simulink model "Modulpruefstand_sim"  (R2024a)
settings: Solver=ode4  StartTime=0.0  StopTime=2  FixedStep=T_A  RelTol=1e-3  EnableMultiTasking=on
values from neighbouring files (symbols this model uses):
  b_Reib = 0    [Modulpruefstand.m]
  g = 9.81    [Modulpruefstand.m]
  I_qstart = 0    [Modulpruefstand.m]
  J = 1.385e-5    (= 1.385e-05)    [Modulpruefstand.m]
  J_Last = m_Last*l_Last^2/(N^2)    (= 0)    [Modulpruefstand.m]
  Ki_I = V_IR/T_In    (= 48205)    [Modulpruefstand.m]
  Ki_omega = V_omegaR/T_omegan    (= 257.626488095)    [Modulpruefstand.m]
  Ki_phi = V_phiR/T_phin    (= 195312.5)    [Modulpruefstand.m]
  Kp_I = V_IR    (= 32.515)    [Modulpruefstand.m]
  Kp_omega = V_omegaR    (= 0.206101190476)    [Modulpruefstand.m]
  Kp_phi = V_phiR    (= 625)    [Modulpruefstand.m]
  l_Last = 0.3    [Modulpruefstand.m]
  L_q = 6.503e-3    (= 0.006503)    [Modulpruefstand.m]
  m_Last = 0    [Modulpruefstand.m]
  Messrauschen = true    [Modulpruefstand.m]
  N = 100    [Modulpruefstand.m]
  n_abs = 2^(17)    (= 131072)    [Modulpruefstand.m]
  n_ink = 11520    [Modulpruefstand.m]
  omega_mstart = 0    [Modulpruefstand.m]
  p = 4    [Modulpruefstand.m]
  phi_mstart = 0    [Modulpruefstand.m]
  psi_PM = 0.028    [Modulpruefstand.m]
  R = 9.641    [Modulpruefstand.m]
  r_abs = 3.77e-5    (= 3.77e-05)    [Modulpruefstand.m]
  r_ink = 1e-5    (= 1e-05)    [Modulpruefstand.m]
  r_strom = 1e-9    (= 1e-09)    [Modulpruefstand.m]
  Signaltyp = 2    [Modulpruefstand.m]
  T_A = 1e-5    (= 1e-05)    [Modulpruefstand.m]
  T_LV = 1e-4    (= 0.0001)    [Modulpruefstand.m]
  T_omegaTP = 10*T_A    (= 0.0001)    [Modulpruefstand.m]
  U_max = 100    [Modulpruefstand.m]
undefined symbols (not defined in the file or in its folder): Kd_strom
libraries: simulink x5, slpidlib x3
settings Model: Creator=ga25cah  LastModifiedBy=75737
settings SolverCC: AlgebraicLoopSolver=TrustRegion
settings DataIOCC: SaveOutput=off  SignalLogging=off  DSMLogging=off  ReturnWorkspaceOutputs=off  TimeSaveName=t_sim
settings DebuggingCC: UnconnectedInputMsg=warning  UnconnectedOutputMsg=warning  UnconnectedLineMsg=warning  ArithmeticOperatorsInVariantConditions=warning
settings ModelReferenceCC: EnableRefExpFcnMdlSchedulingChecks=on
settings SFSimCC: SimUseLocalCustomCode=off  CustomCodeUndefinedFunction=UseInterfaceOnly
settings RTWCC: RTWUseLocalCustomCode=off  GPUComputeCapability=3.5
settings CodeAppCC: StateflowObjectComments=on

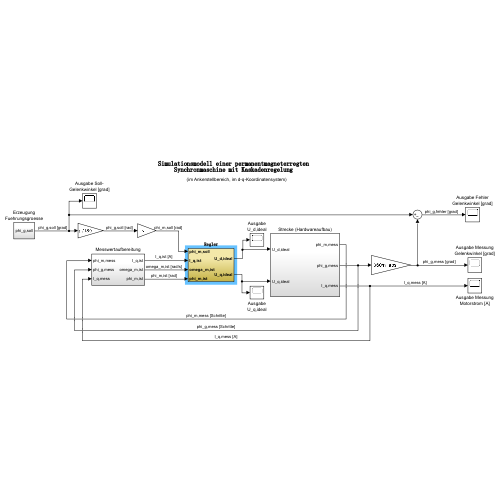
[thumbnail: Simulink's stored preview of the top-level diagram]
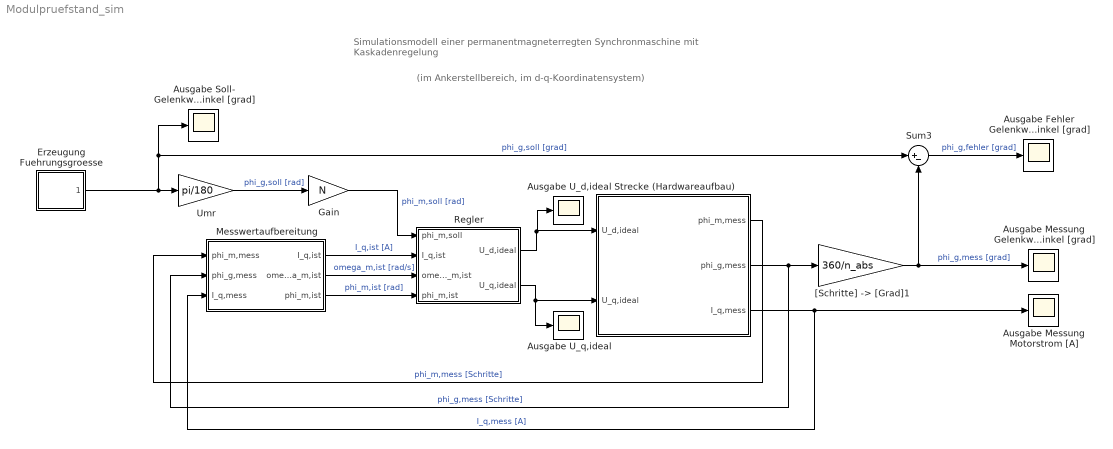
== system Modulpruefstand_sim ==
  note: (im Ankerstellbereich, im d-q-Koordinatensystem)
  note: Simulationsmodell einer permanentmagneterregten
      | Synchronmaschine mit Kaskadenregelung
  Ausgabe U_d,ideal : Scope
  Ausgabe U_q,ideal : Scope
  Ausgabe Fehler Gelenkwinkel [grad] : Scope
  Ausgabe Messung Gelenkwinkel [grad] : Scope
  Ausgabe Messung Motorstrom [A] : Scope
  Ausgabe Soll- Gelenkwinkel [grad] : Scope
  Erzeugung Fuehrungsgroesse : Subsystem
  Gain : Gain  Gain=N
  Messwertaufbereitung : Subsystem
  Regler : Subsystem
  Strecke (Hardwareaufbau) : Subsystem
  Sum3 : Sum  Inputs=|+-
  Umr : Gain  Gain=pi/180
  "[Schritte] -> [Grad]1" : Gain  Gain=360/n_abs
  wires:
  Strecke (Hardwareaufbau)/2(phi_g,mess) -> "[Schritte] -> [Grad]1"/1, Messwertaufbereitung/2(phi_g,mess)  "phi_g,mess [Schritte]"
  Strecke (Hardwareaufbau)/1(phi_m,mess) -> Messwertaufbereitung/1(phi_m,mess)  "phi_m,mess [Schritte]"
  Strecke (Hardwareaufbau)/3(I_q,mess) -> Ausgabe Messung Motorstrom [A]/1, Messwertaufbereitung/3(I_q,mess)  "I_q,mess [A]"
  Regler/2(U_q,ideal) -> Ausgabe U_q,ideal/1, Strecke (Hardwareaufbau)/2(U_q,ideal)
  Messwertaufbereitung/1(I_q,ist) -> Regler/2(I_q,ist)  "I_q,ist [A]"
  Messwertaufbereitung/2(omega_m,ist) -> Regler/3(omega_m,ist)  "omega_m,ist [rad/s]"
  Messwertaufbereitung/3(phi_m,ist) -> Regler/4(phi_m,ist)  "phi_m,ist [rad]"
  Umr/1 -> Gain/1  "phi_g,soll [rad]"
  Regler/1(U_d,ideal) -> Ausgabe U_d,ideal/1, Strecke (Hardwareaufbau)/1(U_d,ideal)
  "[Schritte] -> [Grad]1"/1 -> Ausgabe Messung Gelenkwinkel [grad]/1, Sum3/2  "phi_g,mess [grad]"
  Sum3/1 -> Ausgabe Fehler Gelenkwinkel [grad]/1  "phi_g,fehler [grad]"
  Erzeugung Fuehrungsgroesse/1(phi_g,soll) -> Umr/1, Ausgabe Soll- Gelenkwinkel [grad]/1, Sum3/1  "phi_g,soll [grad]"
  Gain/1 -> Regler/1(phi_m,soll)  "phi_m,soll [rad]"

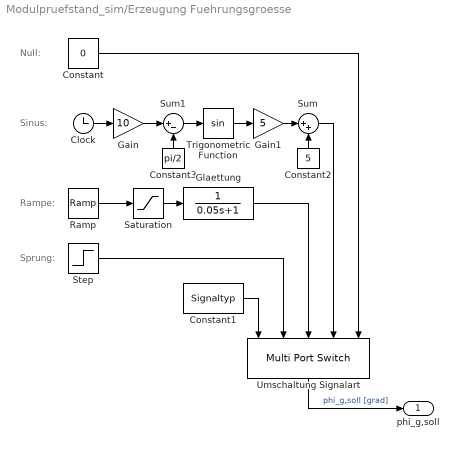
== system Modulpruefstand_sim/Erzeugung Fuehrungsgroesse ==
  note: Sprung:
  note: Rampe:
  note: Sinus:
  note: Null:
  Clock : Clock
  Constant : Constant  Value=0
  Constant1 : Constant  Value=Signaltyp
  Constant2 : Constant  Value=5
  Constant3 : Constant  Value=pi/2
  Gain : Gain  Gain=10
  Gain1 : Gain  Gain=5
  Glaettung : TransferFcn  Denominator=[0.05 1]
  Ramp : simulink/Sources/Ramp  slope=15  start=0.1  InitialOutput=0
  Saturation : Saturate  UpperLimit=15  LowerLimit=0
  Step : Step  Time=0.1  After=15  SampleTime=0
  Sum : Sum  Inputs=|++
  Sum1 : Sum  Inputs=|+-
  Trigonometric Function : Trigonometry
  Umschaltung Signalart : MultiPortSwitch  DataPortForDefault=Additional data port  DiagnosticForDefault=None  SaturateOnIntegerOverflow=off  InputSameDT=off
  phi_g,soll : Outport
  wires:
  Umschaltung Signalart/1 -> phi_g,soll/1  "phi_g,soll [grad]"
  Constant/1 -> Umschaltung Signalart/5
  Constant1/1 -> Umschaltung Signalart/1
  Glaettung/1 -> Umschaltung Signalart/3
  Saturation/1 -> Glaettung/1
  Ramp/1 -> Saturation/1
  Clock/1 -> Gain/1
  Gain/1 -> Sum1/1
  Trigonometric Function/1 -> Gain1/1
  Sum/1 -> Umschaltung Signalart/4
  Step/1 -> Umschaltung Signalart/2
  Gain1/1 -> Sum/1
  Constant2/1 -> Sum/2
  Sum1/1 -> Trigonometric Function/1
  Constant3/1 -> Sum1/2

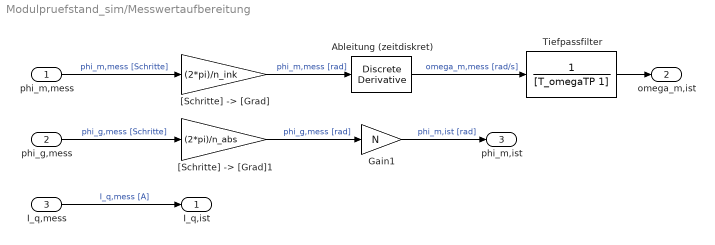
== system Modulpruefstand_sim/Messwertaufbereitung ==
  phi_m,mess : Inport
  phi_g,mess : Inport  Port=2
  I_q,mess : Inport  Port=3
  Ableitung (zeitdiskret) : simulink/Discrete/Discrete Derivative  gainval=1.0  ICPrevScaledInput=0.0  OutMin=[]  OutMax=[]  OutDataType=fixdt(1, 16)  OutScaling=2^-10  DoSatur=off
  Gain1 : Gain  Gain=N
  Tiefpassfilter : TransferFcn  Denominator=[T_omegaTP 1]
  "[Schritte] -> [Grad]" : Gain  Gain=(2*pi)/n_ink
  "[Schritte] -> [Grad]1" : Gain  Gain=(2*pi)/n_abs
  I_q,ist : Outport
  omega_m,ist : Outport  Port=2
  phi_m,ist : Outport  Port=3
  wires:
  phi_m,mess/1 -> "[Schritte] -> [Grad]"/1  "phi_m,mess [Schritte]"
  phi_g,mess/1 -> "[Schritte] -> [Grad]1"/1  "phi_g,mess [Schritte]"
  "[Schritte] -> [Grad]"/1 -> Ableitung (zeitdiskret)/1  "phi_m,mess [rad]"
  "[Schritte] -> [Grad]1"/1 -> Gain1/1  "phi_g,mess [rad]"
  Ableitung (zeitdiskret)/1 -> Tiefpassfilter/1  "omega_m,mess [rad/s]"
  I_q,mess/1 -> I_q,ist/1  "I_q,mess [A]"
  Tiefpassfilter/1 -> omega_m,ist/1
  Gain1/1 -> phi_m,ist/1  "phi_m,ist [rad]"

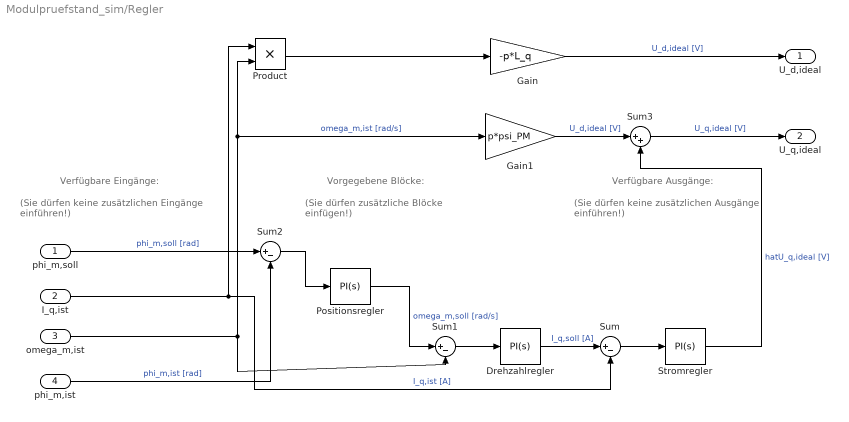
== system Modulpruefstand_sim/Regler ==
  note: (Sie dürfen keine zusätzlichen Eingänge einführen!)
  note: Verfügbare Eingänge:
  note: Vorgegebene Blöcke:
  note: Verfügbare Ausgänge:
  note: (Sie dürfen zusätzliche Blöcke einfügen!)
  note: (Sie dürfen keine zusätzlichen Ausgänge einführen!)
  phi_m,soll : Inport
  I_q,ist : Inport  Port=2
  omega_m,ist : Inport  Port=3
  phi_m,ist : Inport  Port=4
  Drehzahlregler : slpidlib/PID Controller  Controller=PI  Form=Parallel  TimeDomain=Continuous-time  UseExternalTs=off  SampleTime=-1  IntegratorMethod=Forward Euler  FilterMethod=Forward Euler  ControllerParametersSource=internal  P=Kp_omega  I=Ki_omega  UseKiTs=off  D=Kd_strom  UseExternalDerivativeSource=off  N=100  UseFilter=on  TunerSelectOption=Transfer Function Based (PID Tuner App)  InitialConditionSource=internal  InitialConditionForIntegrator=0  InitialConditionForFilter=0  DifferentiatorICPrevScaledInput=0  ExternalReset=none  TrackingMode=off  Kt=1  LimitOutput=off  SatLimitsSource=internal  UpperSaturationLimit=inf  LowerSaturationLimit=-inf  LinearizeAsGain=on  AntiWindupMode=none  Kb=1  LimitIntegrator=off  UpperIntegratorSaturationLimit=inf  LowerIntegratorSaturationLimit=-inf  POutMin=[]  POutMax=[]  IOutMin=[]  IOutMax=[]  DOutMin=[]  DOutMax=[]  NOutMin=[]  NOutMax=[]  SumOutMin=[]  SumOutMax=[]  SaturationOutMin=[]  SaturationOutMax=[]  PParamMin=[]  PParamMax=[]  IParamMin=[]  IParamMax=[]  DParamMin=[]  DParamMax=[]  NParamMin=[]  NParamMax=[]  KbParamMin=[]  KbParamMax=[]  KtParamMin=[]  KtParamMax=[]  KbOutMin=[]  KbOutMax=[]  KtOutMin=[]  KtOutMax=[]  IntegratorOutMin=[]  IntegratorOutMax=[]  FilterOutMin=[]  FilterOutMax=[]  SumI1OutMin=[]  SumI1OutMax=[]  SumI2OutMin=[]  SumI2OutMax=[]  SumI3OutMin=[]  SumI3OutMax=[]  SumI4OutMin=[]  SumI4OutMax=[]  SumDOutMin=[]  SumDOutMax=[]  DifferentiatorOutMin=[]  DifferentiatorOutMax=[]  FilterDiffOutCoefMin=[]  FilterDiffOutCoefMax=[]  ReciprocalOutMin=[]  ReciprocalOutMax=[]  SumDenOutMin=[]  SumDenOutMax=[]  SumNumOutMin=[]  SumNumOutMax=[]  DivideOutMin=[]  DivideOutMax=[]  UdiffTsProdOutMin=[]  UdiffTsProdOutMax=[]  NTsProdOutMin=[]  NTsProdOutMax=[]  UintegralTsProdOutMin=[]  UintegralTsProdOutMax=[]  UngainTsProdOutMin=[]  UngainTsProdOutMax=[]  ClampingZeroOutDataTypeStr=Inherit: Inherit via back propagation  ClampingZeroOutMin=[]  ClampingZeroOutMax=[]  FilterDenConstantOutDataTypeStr=Inherit: Inherit via back propagation  FilterDenConstantOutMin=[]  FilterDenConstantOutMax=[]  PCopyOutDataTypeStr=Inherit: Inherit via back propagation  PCopyOutMin=[]  PCopyOutMax=[]  NCopyOutDataTypeStr=Inherit: Inherit via back propagation  NCopyOutMin=[]  NCopyOutMax=[]  IntegratorContinuousStateAttributes=''  IntegratorStateMustResolveToSignalObject=off  IntegratorRTWStateStorageClass=Auto  FilterContinuousStateAttributes=''  FilterStateMustResolveToSignalObject=off  FilterRTWStateStorageClass=Auto  ParallelPVariant=InternalParameters  IdealPVariant=Disabled  IVariant=InternalParameters  DVariant=Disabled  IntegratorVariant=Continuous  SatVariant=Disabled  AWVariant=Passthrough  PCopyVariant=Disabled  TRVariant=Disabled  FdbkBlocksVariant=Forward  IdealPFdbkVariant=Disabled  SatFdbkVariant=Disabled  DerivativeFilterVariant=Disabled  NVariant=Disabled  NCopyVariant=Disabled_SignalSpec  FilterICVariant=Disabled  IntegratorICVariant=InternalICs  ExternalResetVariant=Disabled  TRSumVariant=Passthrough  SumFdbkVariant=Disabled  SumVariant=Sum_PI  TsampFilterVariant=InternalTs  TsampNgainVariant=Passthrough  TsampIntegralVariant=Disabled_SignalSpec  ExternalSaturationOutDataTypeStr=Inherit: Same as second input  DerivativeSourceVariant=Disabled
  Gain : Gain  Gain=-p*L_q
  Gain1 : Gain  Gain=p*psi_PM
  Positionsregler : slpidlib/PID Controller  Controller=PI  Form=Parallel  TimeDomain=Continuous-time  UseExternalTs=off  SampleTime=-1  IntegratorMethod=Forward Euler  FilterMethod=Forward Euler  ControllerParametersSource=internal  P=Kp_phi  I=Ki_phi  UseKiTs=off  D=0  UseExternalDerivativeSource=off  N=100  UseFilter=on  TunerSelectOption=Transfer Function Based (PID Tuner App)  InitialConditionSource=internal  InitialConditionForIntegrator=0  InitialConditionForFilter=0  DifferentiatorICPrevScaledInput=0  ExternalReset=none  TrackingMode=off  Kt=1  LimitOutput=off  SatLimitsSource=internal  UpperSaturationLimit=inf  LowerSaturationLimit=-inf  LinearizeAsGain=on  AntiWindupMode=none  Kb=1  LimitIntegrator=off  UpperIntegratorSaturationLimit=inf  LowerIntegratorSaturationLimit=-inf  POutMin=[]  POutMax=[]  IOutMin=[]  IOutMax=[]  DOutMin=[]  DOutMax=[]  NOutMin=[]  NOutMax=[]  SumOutMin=[]  SumOutMax=[]  SaturationOutMin=[]  SaturationOutMax=[]  PParamMin=[]  PParamMax=[]  IParamMin=[]  IParamMax=[]  DParamMin=[]  DParamMax=[]  NParamMin=[]  NParamMax=[]  KbParamMin=[]  KbParamMax=[]  KtParamMin=[]  KtParamMax=[]  KbOutMin=[]  KbOutMax=[]  KtOutMin=[]  KtOutMax=[]  IntegratorOutMin=[]  IntegratorOutMax=[]  FilterOutMin=[]  FilterOutMax=[]  SumI1OutMin=[]  SumI1OutMax=[]  SumI2OutMin=[]  SumI2OutMax=[]  SumI3OutMin=[]  SumI3OutMax=[]  SumI4OutMin=[]  SumI4OutMax=[]  SumDOutMin=[]  SumDOutMax=[]  DifferentiatorOutMin=[]  DifferentiatorOutMax=[]  FilterDiffOutCoefMin=[]  FilterDiffOutCoefMax=[]  ReciprocalOutMin=[]  ReciprocalOutMax=[]  SumDenOutMin=[]  SumDenOutMax=[]  SumNumOutMin=[]  SumNumOutMax=[]  DivideOutMin=[]  DivideOutMax=[]  UdiffTsProdOutMin=[]  UdiffTsProdOutMax=[]  NTsProdOutMin=[]  NTsProdOutMax=[]  UintegralTsProdOutMin=[]  UintegralTsProdOutMax=[]  UngainTsProdOutMin=[]  UngainTsProdOutMax=[]  ClampingZeroOutDataTypeStr=Inherit: Inherit via back propagation  ClampingZeroOutMin=[]  ClampingZeroOutMax=[]  FilterDenConstantOutDataTypeStr=Inherit: Inherit via back propagation  FilterDenConstantOutMin=[]  FilterDenConstantOutMax=[]  PCopyOutDataTypeStr=Inherit: Inherit via back propagation  PCopyOutMin=[]  PCopyOutMax=[]  NCopyOutDataTypeStr=Inherit: Inherit via back propagation  NCopyOutMin=[]  NCopyOutMax=[]  IntegratorContinuousStateAttributes=''  IntegratorStateMustResolveToSignalObject=off  IntegratorRTWStateStorageClass=Auto  FilterContinuousStateAttributes=''  FilterStateMustResolveToSignalObject=off  FilterRTWStateStorageClass=Auto  ParallelPVariant=InternalParameters  IdealPVariant=Disabled  IVariant=InternalParameters  DVariant=Disabled  IntegratorVariant=Continuous  SatVariant=Disabled  AWVariant=Passthrough  PCopyVariant=Disabled  TRVariant=Disabled  FdbkBlocksVariant=Forward  IdealPFdbkVariant=Disabled  SatFdbkVariant=Disabled  DerivativeFilterVariant=Disabled  NVariant=Disabled  NCopyVariant=Disabled_SignalSpec  FilterICVariant=Disabled  IntegratorICVariant=InternalICs  ExternalResetVariant=Disabled  TRSumVariant=Passthrough  SumFdbkVariant=Disabled  SumVariant=Sum_PI  TsampFilterVariant=InternalTs  TsampNgainVariant=Passthrough  TsampIntegralVariant=Disabled_SignalSpec  ExternalSaturationOutDataTypeStr=Inherit: Same as second input  DerivativeSourceVariant=Disabled
  Product : Product
  Stromregler : slpidlib/PID Controller  Controller=PI  Form=Parallel  TimeDomain=Continuous-time  UseExternalTs=off  SampleTime=-1  IntegratorMethod=Forward Euler  FilterMethod=Forward Euler  ControllerParametersSource=internal  P=Kp_I  I=Ki_I  UseKiTs=off  D=Kd_strom  UseExternalDerivativeSource=off  N=100  UseFilter=on  TunerSelectOption=Transfer Function Based (PID Tuner App)  InitialConditionSource=internal  InitialConditionForIntegrator=0  InitialConditionForFilter=0  DifferentiatorICPrevScaledInput=0  ExternalReset=none  TrackingMode=off  Kt=1  LimitOutput=off  SatLimitsSource=internal  UpperSaturationLimit=inf  LowerSaturationLimit=-inf  LinearizeAsGain=on  AntiWindupMode=none  Kb=1  LimitIntegrator=off  UpperIntegratorSaturationLimit=inf  LowerIntegratorSaturationLimit=-inf  POutMin=[]  POutMax=[]  IOutMin=[]  IOutMax=[]  DOutMin=[]  DOutMax=[]  NOutMin=[]  NOutMax=[]  SumOutMin=[]  SumOutMax=[]  SaturationOutMin=[]  SaturationOutMax=[]  PParamMin=[]  PParamMax=[]  IParamMin=[]  IParamMax=[]  DParamMin=[]  DParamMax=[]  NParamMin=[]  NParamMax=[]  KbParamMin=[]  KbParamMax=[]  KtParamMin=[]  KtParamMax=[]  KbOutMin=[]  KbOutMax=[]  KtOutMin=[]  KtOutMax=[]  IntegratorOutMin=[]  IntegratorOutMax=[]  FilterOutMin=[]  FilterOutMax=[]  SumI1OutMin=[]  SumI1OutMax=[]  SumI2OutMin=[]  SumI2OutMax=[]  SumI3OutMin=[]  SumI3OutMax=[]  SumI4OutMin=[]  SumI4OutMax=[]  SumDOutMin=[]  SumDOutMax=[]  DifferentiatorOutMin=[]  DifferentiatorOutMax=[]  FilterDiffOutCoefMin=[]  FilterDiffOutCoefMax=[]  ReciprocalOutMin=[]  ReciprocalOutMax=[]  SumDenOutMin=[]  SumDenOutMax=[]  SumNumOutMin=[]  SumNumOutMax=[]  DivideOutMin=[]  DivideOutMax=[]  UdiffTsProdOutMin=[]  UdiffTsProdOutMax=[]  NTsProdOutMin=[]  NTsProdOutMax=[]  UintegralTsProdOutMin=[]  UintegralTsProdOutMax=[]  UngainTsProdOutMin=[]  UngainTsProdOutMax=[]  ClampingZeroOutDataTypeStr=Inherit: Inherit via back propagation  ClampingZeroOutMin=[]  ClampingZeroOutMax=[]  FilterDenConstantOutDataTypeStr=Inherit: Inherit via back propagation  FilterDenConstantOutMin=[]  FilterDenConstantOutMax=[]  PCopyOutDataTypeStr=Inherit: Inherit via back propagation  PCopyOutMin=[]  PCopyOutMax=[]  NCopyOutDataTypeStr=Inherit: Inherit via back propagation  NCopyOutMin=[]  NCopyOutMax=[]  IntegratorContinuousStateAttributes=''  IntegratorStateMustResolveToSignalObject=off  IntegratorRTWStateStorageClass=Auto  FilterContinuousStateAttributes=''  FilterStateMustResolveToSignalObject=off  FilterRTWStateStorageClass=Auto  ParallelPVariant=InternalParameters  IdealPVariant=Disabled  IVariant=InternalParameters  DVariant=Disabled  IntegratorVariant=Continuous  SatVariant=Disabled  AWVariant=Passthrough  PCopyVariant=Disabled  TRVariant=Disabled  FdbkBlocksVariant=Forward  IdealPFdbkVariant=Disabled  SatFdbkVariant=Disabled  DerivativeFilterVariant=Disabled  NVariant=Disabled  NCopyVariant=Disabled_SignalSpec  FilterICVariant=Disabled  IntegratorICVariant=InternalICs  ExternalResetVariant=Disabled  TRSumVariant=Passthrough  SumFdbkVariant=Disabled  SumVariant=Sum_PI  TsampFilterVariant=InternalTs  TsampNgainVariant=Passthrough  TsampIntegralVariant=Disabled_SignalSpec  ExternalSaturationOutDataTypeStr=Inherit: Same as second input  DerivativeSourceVariant=Disabled
  Sum : Sum  Inputs=|+-
  Sum1 : Sum  Inputs=|+-
  Sum2 : Sum  Inputs=|+-
  Sum3 : Sum  Inputs=|++
  U_d,ideal : Outport
  U_q,ideal : Outport  Port=2
  wires:
  Stromregler/1 -> Sum3/2  "hatU_q,ideal [V]"
  omega_m,ist/1 -> Sum1/2, Gain1/1, Product/2  "omega_m,ist [rad/s]"
  Sum3/1 -> U_q,ideal/1  "U_q,ideal [V]"
  phi_m,ist/1 -> Sum2/2  "phi_m,ist [rad]"
  phi_m,soll/1 -> Sum2/1  "phi_m,soll [rad]"
  Gain/1 -> U_d,ideal/1  "U_d,ideal [V]"
  Drehzahlregler/1 -> Sum/1  "I_q,soll [A]"
  I_q,ist/1 -> Sum/2, Product/1  "I_q,ist [A]"
  Positionsregler/1 -> Sum1/1  "omega_m,soll [rad/s]"
  Product/1 -> Gain/1
  Sum/1 -> Stromregler/1
  Sum1/1 -> Drehzahlregler/1
  Sum2/1 -> Positionsregler/1
  Gain1/1 -> Sum3/1  "U_d,ideal [V]"

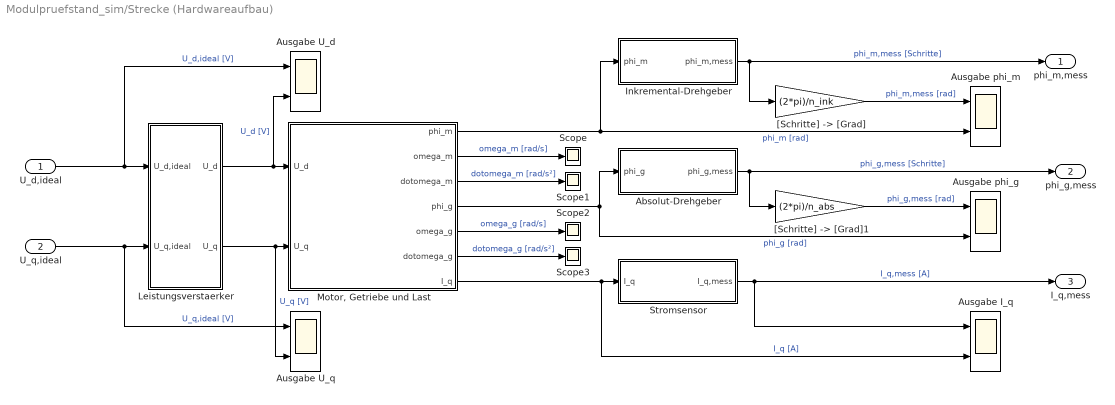
== system Modulpruefstand_sim/Strecke (Hardwareaufbau) ==
  U_d,ideal : Inport
  U_q,ideal : Inport  Port=2
  Absolut-Drehgeber : Subsystem
  Ausgabe I_q : Scope  NumInputPorts=2
  Ausgabe U_d : Scope  NumInputPorts=2
  Ausgabe U_q : Scope  NumInputPorts=2
  Ausgabe phi_g : Scope  NumInputPorts=2
  Ausgabe phi_m : Scope  NumInputPorts=2
  Inkremental-Drehgeber : Subsystem
  Leistungsverstaerker : Subsystem
  "Motor, Getriebe und Last" : Subsystem
  Scope{,1..3} (4 alike) : Scope
  Stromsensor : Subsystem
  "[Schritte] -> [Grad]" : Gain  Gain=(2*pi)/n_ink
  "[Schritte] -> [Grad]1" : Gain  Gain=(2*pi)/n_abs
  phi_m,mess : Outport
  phi_g,mess : Outport  Port=2
  I_q,mess : Outport  Port=3
  wires:
  "Motor, Getriebe und Last"/7(I_q) -> Ausgabe I_q/2, Stromsensor/1(I_q)  "I_q [A]"
  Stromsensor/1(I_q,mess) -> Ausgabe I_q/1, I_q,mess/1  "I_q,mess [A]"
  "Motor, Getriebe und Last"/1(phi_m) -> Ausgabe phi_m/2, Inkremental-Drehgeber/1(phi_m)  "phi_m [rad]"
  "Motor, Getriebe und Last"/4(phi_g) -> Absolut-Drehgeber/1(phi_g), Ausgabe phi_g/2  "phi_g [rad]"
  Inkremental-Drehgeber/1(phi_m,mess) -> phi_m,mess/1, "[Schritte] -> [Grad]"/1  "phi_m,mess [Schritte]"
  Absolut-Drehgeber/1(phi_g,mess) -> "[Schritte] -> [Grad]1"/1, phi_g,mess/1  "phi_g,mess [Schritte]"
  U_d,ideal/1 -> Leistungsverstaerker/1(U_d,ideal), Ausgabe U_d/1  "U_d,ideal [V]"
  Leistungsverstaerker/1(U_d) -> Ausgabe U_d/2, "Motor, Getriebe und Last"/1(U_d)  "U_d [V]"
  "Motor, Getriebe und Last"/2(omega_m) -> Scope/1  "omega_m [rad/s]"
  "Motor, Getriebe und Last"/3(dotomega_m) -> Scope1/1  "dotomega_m [rad/s²]"
  "Motor, Getriebe und Last"/5(omega_g) -> Scope2/1  "omega_g [rad/s]"
  U_q,ideal/1 -> Ausgabe U_q/1, Leistungsverstaerker/2(U_q,ideal)  "U_q,ideal [V]"
  Leistungsverstaerker/2(U_q) -> Ausgabe U_q/2, "Motor, Getriebe und Last"/2(U_q)  "U_q [V]"
  "Motor, Getriebe und Last"/6(dotomega_g) -> Scope3/1  "dotomega_g [rad/s²]"
  "[Schritte] -> [Grad]"/1 -> Ausgabe phi_m/1  "phi_m,mess [rad]"
  "[Schritte] -> [Grad]1"/1 -> Ausgabe phi_g/1  "phi_g,mess [rad]"

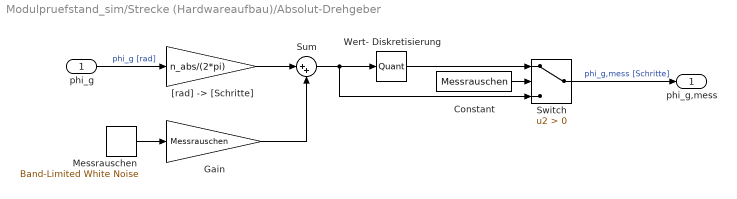
== system Modulpruefstand_sim/Strecke (Hardwareaufbau)/Absolut-Drehgeber ==
  phi_g : Inport
  Constant : Constant  Value=Messrauschen
  Gain : Gain  Gain=Messrauschen
  Messrauschen : simulink/Sources/Band-Limited White Noise  Cov=[r_abs]  Ts=T_A  seed=[23341]
  Sum : Sum  Inputs=|++
  Switch : Switch  Criteria=u2 > Threshold  SaturateOnIntegerOverflow=off  InputSameDT=off
  Wert- Diskretisierung : Quantizer  QuantizationInterval=1
  "[rad] -> [Schritte]" : Gain  Gain=n_abs/(2*pi)
  phi_g,mess : Outport
  wires:
  phi_g/1 -> "[rad] -> [Schritte]"/1  "phi_g [rad]"
  Switch/1 -> phi_g,mess/1  "phi_g,mess [Schritte]"
  "[rad] -> [Schritte]"/1 -> Sum/1
  Messrauschen/1 -> Gain/1
  Wert- Diskretisierung/1 -> Switch/1
  Sum/1 -> Wert- Diskretisierung/1, Switch/3
  Constant/1 -> Switch/2
  Gain/1 -> Sum/2

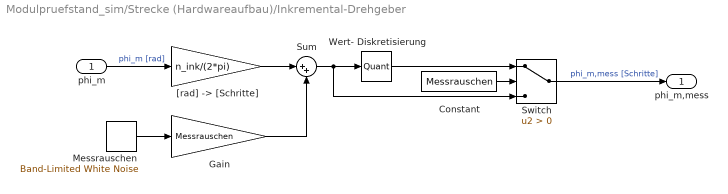
== system Modulpruefstand_sim/Strecke (Hardwareaufbau)/Inkremental-Drehgeber ==
  phi_m : Inport
  Constant : Constant  Value=Messrauschen
  Gain : Gain  Gain=Messrauschen
  Messrauschen : simulink/Sources/Band-Limited White Noise  Cov=[r_ink]  Ts=T_A  seed=[23341]
  Sum : Sum  Inputs=|++
  Switch : Switch  Criteria=u2 > Threshold  SaturateOnIntegerOverflow=off  InputSameDT=off
  Wert- Diskretisierung : Quantizer  QuantizationInterval=1
  "[rad] -> [Schritte]" : Gain  Gain=n_ink/(2*pi)
  phi_m,mess : Outport
  wires:
  phi_m/1 -> "[rad] -> [Schritte]"/1  "phi_m [rad]"
  Wert- Diskretisierung/1 -> Switch/1
  Messrauschen/1 -> Gain/1
  "[rad] -> [Schritte]"/1 -> Sum/1
  Sum/1 -> Switch/3, Wert- Diskretisierung/1
  Switch/1 -> phi_m,mess/1  "phi_m,mess [Schritte]"
  Constant/1 -> Switch/2
  Gain/1 -> Sum/2

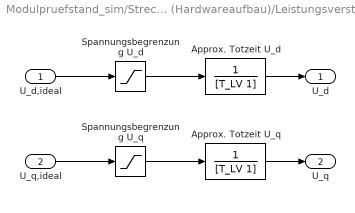
== system Modulpruefstand_sim/Strecke (Hardwareaufbau)/Leistungsverstaerker ==
  U_d,ideal : Inport
  U_q,ideal : Inport  Port=2
  Approx. Totzeit U_d : TransferFcn  Denominator=[T_LV 1]
  Approx. Totzeit U_q : TransferFcn  Denominator=[T_LV 1]
  Spannungsbegrenzung U_d : Saturate  UpperLimit=U_max  LowerLimit=-U_max
  Spannungsbegrenzung U_q : Saturate  UpperLimit=U_max  LowerLimit=-U_max
  U_d : Outport
  U_q : Outport  Port=2
  wires:
  Spannungsbegrenzung U_d/1 -> Approx. Totzeit U_d/1
  U_d,ideal/1 -> Spannungsbegrenzung U_d/1
  Spannungsbegrenzung U_q/1 -> Approx. Totzeit U_q/1
  U_q,ideal/1 -> Spannungsbegrenzung U_q/1
  Approx. Totzeit U_d/1 -> U_d/1
  Approx. Totzeit U_q/1 -> U_q/1

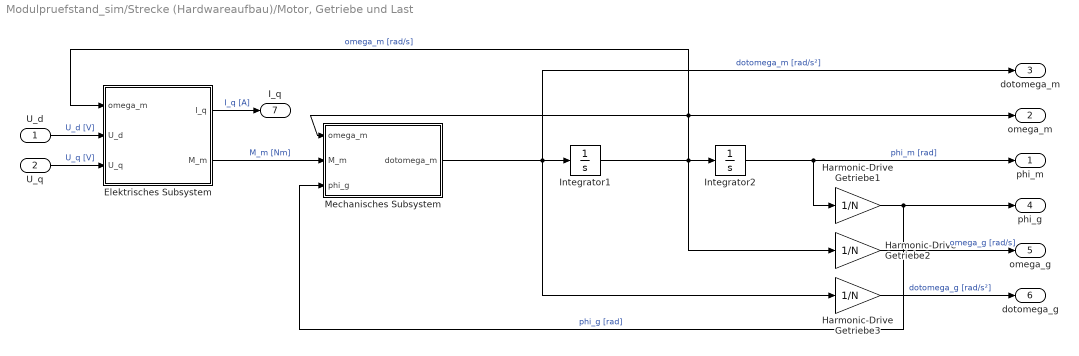
== system Modulpruefstand_sim/Strecke (Hardwareaufbau)/Motor, Getriebe und Last ==
  U_d : Inport
  U_q : Inport  Port=2
  Elektrisches Subsystem : Subsystem
  Harmonic-Drive Getriebe1 : Gain  Gain=1/N
  Harmonic-Drive Getriebe2 : Gain  Gain=1/N
  Harmonic-Drive Getriebe3 : Gain  Gain=1/N
  Integrator1 : Integrator  InitialCondition=omega_mstart
  Integrator2 : Integrator  InitialCondition=phi_mstart
  Mechanisches Subsystem : Subsystem
  phi_m : Outport
  omega_m : Outport  Port=2
  dotomega_m : Outport  Port=3
  phi_g : Outport  Port=4
  omega_g : Outport  Port=5
  dotomega_g : Outport  Port=6
  I_q : Outport  Port=7
  wires:
  Integrator1/1 -> Mechanisches Subsystem/1(omega_m), Elektrisches Subsystem/1(omega_m), omega_m/1, Harmonic-Drive Getriebe2/1, Integrator2/1  "omega_m [rad/s]"
  Integrator2/1 -> phi_m/1, Harmonic-Drive Getriebe1/1  "phi_m [rad]"
  Harmonic-Drive Getriebe2/1 -> omega_g/1  "omega_g [rad/s]"
  Harmonic-Drive Getriebe3/1 -> dotomega_g/1  "dotomega_g [rad/s²]"
  Harmonic-Drive Getriebe1/1 -> Mechanisches Subsystem/3(phi_g), phi_g/1  "phi_g [rad]"
  Elektrisches Subsystem/1(I_q) -> I_q/1  "I_q [A]"
  U_d/1 -> Elektrisches Subsystem/2(U_d)  "U_d [V]"
  U_q/1 -> Elektrisches Subsystem/3(U_q)  "U_q [V]"
  Mechanisches Subsystem/1(dotomega_m) -> Harmonic-Drive Getriebe3/1, dotomega_m/1, Integrator1/1  "dotomega_m [rad/s²]"
  Elektrisches Subsystem/2(M_m) -> Mechanisches Subsystem/2(M_m)  "M_m [Nm]"

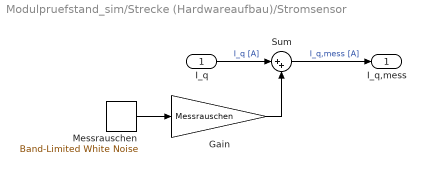
== system Modulpruefstand_sim/Strecke (Hardwareaufbau)/Stromsensor ==
  I_q : Inport
  Gain : Gain  Gain=Messrauschen
  Messrauschen : simulink/Sources/Band-Limited White Noise  Cov=[r_strom]  Ts=T_A  seed=[23341]
  Sum : Sum  Inputs=|++
  I_q,mess : Outport
  wires:
  I_q/1 -> Sum/1  "I_q [A]"
  Sum/1 -> I_q,mess/1  "I_q,mess [A]"
  Messrauschen/1 -> Gain/1
  Gain/1 -> Sum/2

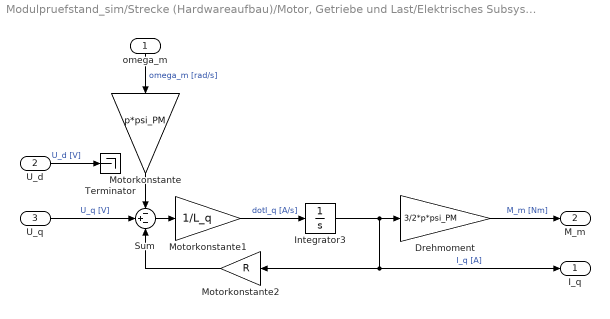
== system Modulpruefstand_sim/Strecke (Hardwareaufbau)/Motor, Getriebe und Last/Elektrisches Subsystem ==
  omega_m : Inport
  U_d : Inport  Port=2
  U_q : Inport  Port=3
  Drehmoment : Gain  Gain=3/2*p*psi_PM
  Integrator3 : Integrator  InitialCondition=I_qstart
  Motorkonstante : Gain  Gain=p*psi_PM
  Motorkonstante1 : Gain  Gain=1/L_q
  Motorkonstante2 : Gain  Gain=R
  Sum : Sum  Inputs=-+-
  Terminator : Terminator
  I_q : Outport
  M_m : Outport  Port=2
  wires:
  omega_m/1 -> Motorkonstante/1  "omega_m [rad/s]"
  Motorkonstante2/1 -> Sum/3
  Drehmoment/1 -> M_m/1  "M_m [Nm]"
  Motorkonstante1/1 -> Integrator3/1  "dotI_q [A/s]"
  Sum/1 -> Motorkonstante1/1
  Motorkonstante/1 -> Sum/1
  Integrator3/1 -> Drehmoment/1, Motorkonstante2/1, I_q/1  "I_q [A]"
  U_q/1 -> Sum/2  "U_q [V]"
  U_d/1 -> Terminator/1  "U_d [V]"

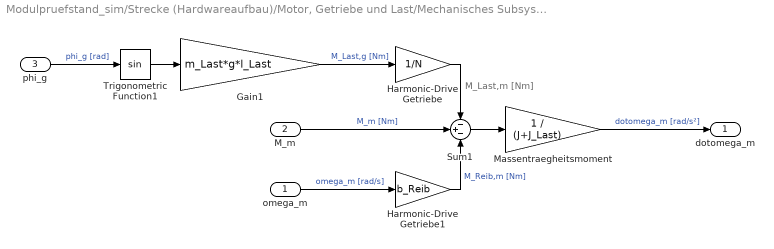
== system Modulpruefstand_sim/Strecke (Hardwareaufbau)/Motor, Getriebe und Last/Mechanisches Subsystem ==
  note: M_Last,m [Nm]
  omega_m : Inport
  M_m : Inport  Port=2
  phi_g : Inport  Port=3
  Gain1 : Gain  Gain=m_Last*g*l_Last
  Harmonic-Drive Getriebe : Gain  Gain=1/N
  Harmonic-Drive Getriebe1 : Gain  Gain=b_Reib
  Massentraegheitsmoment : Gain  Gain=1 / (J+J_Last)
  Sum1 : Sum  Inputs=-+-
  Trigonometric Function1 : Trigonometry
  dotomega_m : Outport
  wires:
  Trigonometric Function1/1 -> Gain1/1
  Sum1/1 -> Massentraegheitsmoment/1
  Massentraegheitsmoment/1 -> dotomega_m/1  "dotomega_m [rad/s²]"
  M_m/1 -> Sum1/2  "M_m [Nm]"
  phi_g/1 -> Trigonometric Function1/1  "phi_g [rad]"
  Gain1/1 -> Harmonic-Drive Getriebe/1  "M_Last,g [Nm]"
  Harmonic-Drive Getriebe/1 -> Sum1/1
  omega_m/1 -> Harmonic-Drive Getriebe1/1  "omega_m [rad/s]"
  Harmonic-Drive Getriebe1/1 -> Sum1/3  "M_Reib,m [Nm]"
